simulink model "test_FAST_qLPVMPC"  (R2023a)
settings: Solver=FixedStepAuto  StartTime=0.0  StopTime=400  FixedStep=DT  RelTol=1e-3
values from neighbouring files (symbols this model uses):
  Lin_points : value not decoded    [DD_test.sldd]
undefined symbols (not defined in the file or in its folder): Rotor_Lambda
settings Model: DataDictionary=DD_test.sldd  ExtModeTrigMode=oneshot  Creator=Hazim Namik  LastModifiedBy=ditt_aj
settings SolverCC: AlgebraicLoopSolver=TrustRegion
settings DataIOCC: LimitDataPoints=on  SaveFormat=Array  ReturnWorkspaceOutputs=off
settings OptimizationCC: BlockReduction=off  BooleanDataType=off  LifeSpan=inf
settings DebuggingCC: SaveWithParameterizedLinksMsg=none  UnderspecifiedInitializationDetection=Classic  MergeDetectMultiDrivingBlocksExec=none  SignalResolutionControl=TryResolveAllWithWarning  UnconnectedInputMsg=warning  UnconnectedOutputMsg=warning  UnconnectedLineMsg=warning  SFUnexpectedBacktrackingDiag=warning  SFNoUnconditionalDefaultTransitionDiag=warning  SFExecutionAtInitializationDiag=none  ArithmeticOperatorsInVariantConditions=warning
settings HardwareCC: ProdBitPerPointer=32  ProdBitPerSizeT=32  ProdBitPerPtrDiffT=32  ProdLargestAtomicFloat=None  ProdIntDivRoundTo=Undefined  ProdEndianess=Unspecified  ProdWordSize=32  ProdHWDeviceType=32-bit Generic  TargetUnknown=on
settings ModelReferenceCC: EnableRefExpFcnMdlSchedulingChecks=on  PropagateSignalLabelsOutOfModel=off
settings SFSimCC: SimUseLocalCustomCode=off  CustomCodeUndefinedFunction=UseInterfaceOnly
settings RTWCC: RTWUseLocalCustomCode=off  DLArmComputeVersion=19.05
settings CodeAppCC: StateflowObjectComments=on
settings GRTTargetCC: TargetLangStandard=C89/C90 (ANSI)
settings ConfigComp: CovMetricSettings=dw  CovSaveCumulativeToWorkspaceVar=on  CovSaveSingleToWorkspaceVar=on  CovExternalEMLEnable=off

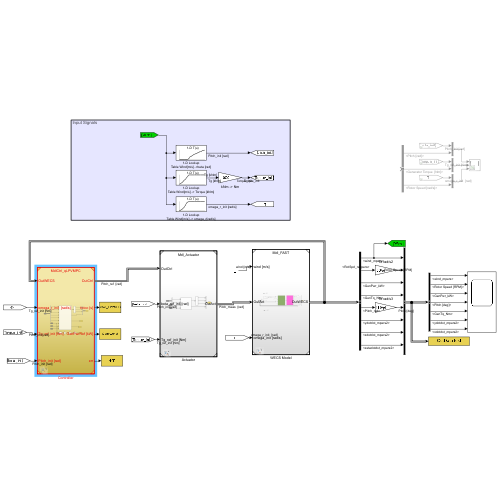
[thumbnail: Simulink's stored preview of the top-level diagram]
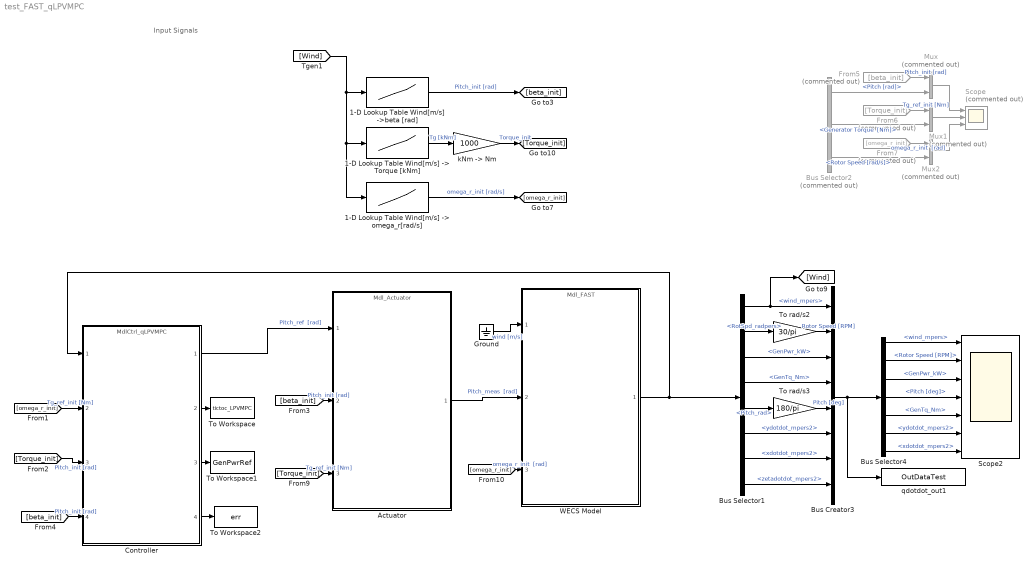
== system test_FAST_qLPVMPC ==
  note: Input Signals
  "1-D Lookup Table Wind[m/s] -> Torque [kNm]" : Lookup_n-D  NumberOfTableDimensions=1  BreakpointsForDimension1=Lin_points.V  BreakpointsForDimension2=Rotor_Lambda  Table=Lin_points.Torque  InternalRulePriority=Speed  RndMeth=Simplest
  "1-D Lookup Table Wind[m/s] -> omega_r[rad/s]" : Lookup_n-D  NumberOfTableDimensions=1  BreakpointsForDimension1=Lin_points.V  BreakpointsForDimension2=Rotor_Lambda  Table=Lin_points.RSpeed  InternalRulePriority=Speed  RndMeth=Simplest
  1-D Lookup Table Wind[m/s] ->beta [rad] : Lookup_n-D  NumberOfTableDimensions=1  BreakpointsForDimension1=Lin_points.V  BreakpointsForDimension2=Rotor_Lambda  Table=Lin_points.Pitch  InternalRulePriority=Speed  RndMeth=Simplest
  Actuator : ModelReference  ModelNameDialog=Mdl_Actuator.slx  SimulationMode=Normal  ModelReferenceVersion=7.0
  Bus Creator3 : BusCreator  Inputs=8
  Bus Selector1 : BusSelector  OutputSignals=wind_mpers,RotSpd_radpers,GenPwr_kW,GenTq_Nm,Pitch_rad,ydotdot_mpers2,xdotdot_mpers2,zetadotdot_mpers2
  Bus Selector2 : BusSelector  Commented=on  OutputSignals="Pitch [rad],Generator Torque  [Nm],Rotor Speed [rad/s]"
  Bus Selector4 : BusSelector  OutputSignals=wind_mpers,Rotor Speed [RPM],GenPwr_kW,Pitch [deg],GenTq_Nm,ydotdot_mpers2,xdotdot_mpers2
  Controller : ModelReference  ModelNameDialog=MdlCtrl_qLPVMPC.slx  SimulationMode=Normal  ModelReferenceVersion=7.30
  From5 : From  Commented=on  GotoTag=beta_init
      settings: CloseFcn=tagdialog Close
  From6 : From  Commented=on  GotoTag=Torque_init
      settings: CloseFcn=tagdialog Close
  From7 : From  Commented=on  GotoTag=omega_r_init
      settings: CloseFcn=tagdialog Close
  Ground : Ground
  Mux : Mux  Commented=on  Inputs=2
  Mux1 : Mux  Commented=on  Inputs=2
  Mux2 : Mux  Commented=on  Inputs=2
  Scope : Scope  Commented=on  NumInputPorts=3
  Scope2 : Scope  NumInputPorts=7
      settings: Tag=Scope
  To Workspace : ToWorkspace  VariableName=tictoc_LPVMPC  SaveFormat=Timeseries  SampleTime=-1
  To Workspace1 : ToWorkspace  VariableName=GenPwrRef  SaveFormat=Timeseries  SampleTime=-1
  To Workspace2 : ToWorkspace  VariableName=err  SaveFormat=Timeseries  SampleTime=-1
  To rad/s2 : Gain  Gain=30/pi
  To rad/s3 : Gain  Gain=180/pi
  WECS Model : ModelReference  ModelNameDialog=Mdl_FAST.slx  SimulationMode=Normal  ModelReferenceVersion=8.0
  "kNm -> Nm" : Gain  Gain=1000
  qdotdot_out1 : ToWorkspace  VariableName=OutDataTest  SampleTime=-1
  wires:
  [Torque_init] -> Actuator/3  "Tg_ref_init [Nm]"
  "1-D Lookup Table Wind[m/s] -> Torque [kNm]"/1 -> "kNm -> Nm"/1  "Tg [kNm]"
  "1-D Lookup Table Wind[m/s] -> omega_r[rad/s]"/1 -> [omega_r_init]  "omega_r_init [rad/s]"
  Actuator/1 -> WECS Model/2  "Pitch_meas  [rad]"
  Ground/1 -> WECS Model/1  "wind [m/s]"
  [Wind] -> "1-D Lookup Table Wind[m/s] -> omega_r[rad/s]"/1, "1-D Lookup Table Wind[m/s] -> Torque [kNm]"/1, 1-D Lookup Table Wind[m/s] ->beta [rad]/1
  "kNm -> Nm"/1 -> [Torque_init]  "Torque_init"
  1-D Lookup Table Wind[m/s] ->beta [rad]/1 -> [beta_init]  "Pitch_init [rad]"
  [omega_r_init] -> WECS Model/3  "omega_r_init  [rad]"
  Mux/1 -> Scope/1
  From5/1 -> Mux/1  "Pitch_init [rad]"
  Mux1/1 -> Scope/2
  Mux2/1 -> Scope/3
  From6/1 -> Mux1/1  "Tg_ref_init [Nm]"
  From7/1 -> Mux2/1  "omega_r_init  [rad]"
  Bus Selector2/1 -> Mux/2  "<Pitch [rad]>"
  Bus Selector2/2 -> Mux1/2  "<Generator Torque  [Nm]>"
  Bus Selector2/3 -> Mux2/2  "<Rotor Speed [rad/s]>"
  Controller/1 -> Actuator/1  "Pitch_ref  [rad]"
  [beta_init] -> Actuator/2  "Pitch_init [rad]"
  Bus Selector4/1 -> Scope2/1  "<wind_mpers>"
  Bus Selector1/5 -> To rad/s3/1  "<Pitch_rad>"
  Bus Selector1/2 -> To rad/s2/1  "<RotSpd_radpers>"
  Bus Selector1/3 -> Bus Creator3/3  "<GenPwr_kW>"
  Bus Creator3/1 -> Bus Selector4/1, qdotdot_out1/1
  WECS Model/1 -> Controller/1, Bus Selector1/1
  To rad/s3/1 -> Bus Creator3/5  "Pitch [deg]"
  Bus Selector4/2 -> Scope2/2  "<Rotor Speed [RPM]>"
  Bus Selector4/6 -> Scope2/6  "<ydotdot_mpers2>"
  Bus Selector1/1 -> [Wind], Bus Creator3/1  "<wind_mpers>"
  Bus Selector4/5 -> Scope2/5  "<GenTq_Nm>"
  Bus Selector4/7 -> Scope2/7  "<xdotdot_mpers2>"
  Bus Selector1/4 -> Bus Creator3/4  "<GenTq_Nm>"
  To rad/s2/1 -> Bus Creator3/2  "Rotor Speed [RPM]"
  Bus Selector4/4 -> Scope2/4  "<Pitch [deg]>"
  Bus Selector1/8 -> Bus Creator3/8  "<zetadotdot_mpers2>"
  Bus Selector4/3 -> Scope2/3  "<GenPwr_kW>"
  Bus Selector1/7 -> Bus Creator3/7  "<xdotdot_mpers2>"
  Bus Selector1/6 -> Bus Creator3/6  "<ydotdot_mpers2>"
  Controller/4 -> To Workspace2/1
  Controller/3 -> To Workspace1/1
  Controller/2 -> To Workspace/1
  [beta_init] -> Controller/4  "Pitch_init [rad]"
  [omega_r_init] -> Controller/2  "Tg_ref_init [Nm]"
  [Torque_init] -> Controller/3  "Pitch_init [rad]"
